simulink model "Vehicle_Dynamics_Testrig"  (R2025a)
settings: Solver=ode23t  StartTime=0.0  StopTime=400  RelTol=1e-3  AbsTol=1e-4  EnableMultiTasking=on
PostLoadFcn:
  | warning off Simulink:Engine:SaveWithDisabledLinks_Warning
  | warning off Simulink:Engine:UsingDefaultMaxStepSize
undefined symbols (not defined in the file): DCT_Param, sigbuilder_block
libraries: fl_lib x22, nesl_utility x6, DCT_Vehicle_Dynamics_Lib x1, sdl_lib x1
Description:
  | Copyright 2014-2025 The MathWorks, Inc.
settings Model: Creator=smiller  LastModifiedBy=smiller
settings SolverCC: AutoScaleAbsTol=off  AlgebraicLoopSolver=TrustRegion
settings DataIOCC: LimitDataPoints=on  SaveFormat=Array  SignalLoggingSaveFormat=ModelDataLogs  ReturnWorkspaceOutputs=off
settings OptimizationCC: ReuseModelBlockBuffer=off  ExpressionDepthLimit=2147483647.0  LifeSpan=inf
settings DebuggingCC: UnderspecifiedInitializationDetection=Classic  MergeDetectMultiDrivingBlocksExec=none  SolverPrmCheckMsg=warning  FcnCallInpInsideContextMsg=warning  UnconnectedInputMsg=warning  UnconnectedOutputMsg=warning  UnconnectedLineMsg=warning  AllowSymbolicDim=off  StateNameClashWarn=warning  PregeneratedLibrarySubsystemCodeDiagnostic=none  SFUnexpectedBacktrackingDiag=warning  SFNoUnconditionalDefaultTransitionDiag=warning  SFExecutionAtInitializationDiag=none  ArithmeticOperatorsInVariantConditions=warning
settings HardwareCC: ProdBitPerPointer=32.0  ProdBitPerSizeT=32.0  ProdBitPerPtrDiffT=32.0  ProdLargestAtomicFloat=None  ProdIntDivRoundTo=Undefined  ProdEndianess=Unspecified  ProdWordSize=32.0  ProdHWDeviceType=32-bit Generic
settings ModelReferenceCC: EnableRefExpFcnMdlSchedulingChecks=on  PropagateSignalLabelsOutOfModel=off
settings SFSimCC: SimUseLocalCustomCode=off  CustomCodeUndefinedFunction=UseInterfaceOnly
settings RTWCC: RTWUseLocalCustomCode=off  GPUComputeCapability=3.5  DLArmComputeVersion=19.05
settings CodeAppCC: StateflowObjectComments=on
settings GRTTargetCC: TargetLangStandard=C89/C90 (ANSI)  CombineOutputUpdateFcns=off  GRTInterface=on
settings ConfigComp: CovMetricSettings=dw  CovSaveCumulativeToWorkspaceVar=on  CovSaveSingleToWorkspaceVar=on  CovExternalEMLEnable=off  CovSFcnEnable=off
settings SimscapeCC: SimscapeNormalizeSystem=off  SimscapeNominalValues="[{\"value\":\"10\",\"unit\":\"V\"},{\"value\":\"1\",\"unit\":\"A\"},{\"value\":\"10\",\"unit\":\"N*m\"},{\"value\":\"10\",\"unit\":\"bar\"},{\"value\":\"100\",\"unit\":\"kJ/kg\"},{\"value\":\"1\",\"unit\":\"kW\"},{\"value\":\"300\",\"unit\":\"K\"},{\"value\":\"100\",\"unit\":\"cm^3/s\"},{\"value\":\"1\",\"unit\":\"kN\"},{\"value\":\"1\",\"unit\":\"g/cm^3\"},{\"value\":\"1\",\"unit\":\"l\"},{\"value\":\"1\",\"unit\":\"cm^2\"},{\"value\":\"60\",\"unit\":\"Hz\"}]"

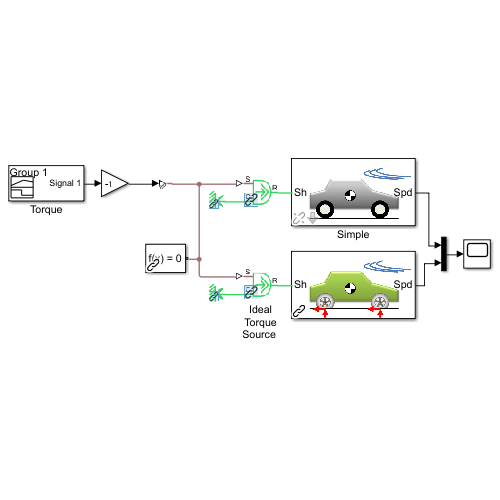
[thumbnail: Simulink's stored preview of the top-level diagram]
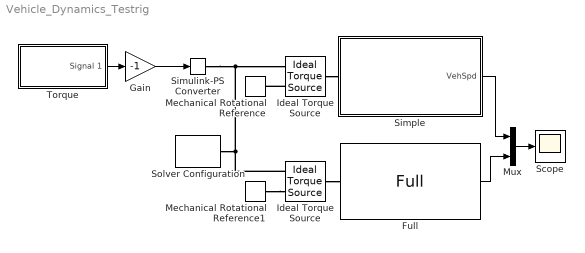
== system Vehicle_Dynamics_Testrig ==
  Full : DCT_Vehicle_Dynamics_Lib/Full  SystemSampleTime=-1  VariantActivationTime=update diagram  EmptyChoice=off  PassThrough=off  PassThroughVariantControl=(default)  EmptyChoiceVariantControl=(default)  AllowFlexibleInterface=on  Latency=0  AutoFrameSizeCalculation=off
  Gain : Gain  Gain=-1
  Ideal Torque Source : fl_lib/Mechanical/Mechanical Sources/Ideal Torque Source
  "Ideal Torque Source " : fl_lib/Mechanical/Mechanical Sources/Ideal Torque Source
  Mechanical Rotational Reference : fl_lib/Mechanical/Rotational Elements/Mechanical Rotational Reference
  Mechanical Rotational Reference1 : fl_lib/Mechanical/Rotational Elements/Mechanical Rotational Reference
  Mux : Mux  Inputs=2
  Scope : Scope
      settings: TimeSpan=400  ActiveDisplayYMinimum=-12.14127  ActiveDisplayYMaximum=109.27138
  Simple : Subsystem  AncestorBlock=DCT_Vehicle_Dynamics_Lib/Simple  mask(Rigid vehicle model){mass=DCT_Param.Vehicle.Mass, area=DCT_Param.Vehicle.Frontal_Area, Cd=DCT_Param.Vehicle.Aero_Drag_Coeff, radius=DCT_Param.Vehicle.Tire.Radius, wheel_inertia=DCT_Param.Vehicle.Tire.Inertia, gear_ratio=DCT_Param.Vehicle.Final_Drive_Ratio}
      mask prompts: mass "Vehicle mass (Kg)"; area "Vehicle Area (m^2)"; Cd "Aerodynamic drag coefficient (unitless)"; radius "Tire radius (m)"; wheel_inertia "Total wheel inertia (kg*m^2)"; gear_ratio "Engine to vehicle gear ratio"
      mask help: Model vehicle effective inertia and drag force as seen by the engine. It is assumed that the vehicle is moving on flat terrain. No bearing friction or gear losses are included.
      mask init:
      | gravity = 9.81;
      settings: LibrarySourceBlock=DCT_Vehicle_Dynamics_Lib/Simple
      mask Display:
      | image(imread('DCT_Vehicle_Dynamics_Simple_IMAGE.jpg'));
      | port_label('LConn',1,'Sh');
      | port_label('output',1,'Spd');
  Simulink-PS Converter : nesl_utility/Simulink-PS Converter  PhysicalDomain=network_engine_domain  SubClassName=ps_input  LeftPortType=input  RightPortType=output  PseudoPeriodic=off  Frequencies=[]  NoiseDistribution=none  NoiseParameters=[]  Unit=1  AffineConversion=off  FilteringAndDerivatives=zero  SimscapeFilterOrder=1  InputFilterTimeConstant=0.005  UdotUserProvided=0
  Solver Configuration : nesl_utility/Solver Configuration  PhysicalDomain=network_engine_domain  SubClassName=solver  LeftPortType=input  RightPortType=generic  Tones=[]  Harmonics=[]  SimulateNoise=off  Profile=off  UseLocalSampling=off  EnableSwitchedLinearOptims=on  FrequencyDomain=off  UseCCode=off  RelTol=0.001  AbsTol=1e-06  MinStep=1e-09  ToWorkspace=off  RevertToSquareIcSolve=off  NumHomotopyIterations=100  PhasorMode=off  PhasorModeNumHarmonics=1  ConsistencySolver=NEWTON_FTOL  IndexReductionMethod=DerivativeReplacement  DoDC=off  ResidualTolerance=1e-9  ConsistencyTolSource=GLOBAL  ConsistencyAbsTol=0.001  ConsistencyRelTol=0.001  ConsistencyTolFactor=0.001  UseLocalSolver=off  LocalSolverChoice=NE_BACKWARD_EULER_ADVANCER  ResolveIndetEquations=on  FunctionEvalNumThread=1  LocalSolverSampleTime=.001  DoFixedCost=off  MaxNonlinIter=3  MaxModeIter=2  ComputeImpulses=off  ImpulseIterations=2  LinearAlgebra=Sparse  LinearAlgebraNumThread=0  EquationFormulation=NE_TIME_EF  DelaysMemoryBudget=1024  AutomaticFiltering=on  FilteringTimeConstant=0.001  PartitionStorageMethod=AS_NEEDED  PartitionMemoryBudget=1024  PartitionMethod=FAST  MultibodyUseLocalSolver=off  MultibodyLocalSolverChoice=ODE1  MultibodyLocalSolverSampleTime=0.001
  Torque : Subsystem  Tag=STV Subsys  LoadFcn=sigbuilder_block('load');  StartFcn=sigbuilder_block('start');  StopFcn=sigbuilder_block('stop');  ClipboardFcn=sigbuilder_block('clipboard');  mask(Sigbuilder block){tuvar=[0:10]}
      mask help: Create and generate interchangeable groups of signals whose waveforms are piecewise linear.
      mask init:
      | if ~strcmp(get_param(bdroot(gcbh),'SimulationStatus'),'stopped') tuvar = sigbuilder_block('maskInit'); end
      settings: CopyFcn=sigbuilder_block('copy');  DeleteFcn=sigbuilder_block('delete');  ModelCloseFcn=sigbuilder_block('modelClose');  PreSaveFcn=sigbuilder_block('preSave');  PauseFcn=sigbuilder_block('pause')  ContinueFcn=sigbuilder_block('continue')  NameChangeFcn=sigbuilder_block('namechange');  OpenFcn=sigbuilder_block('open',[437.25 199.5 550.5 399.75 ]);  CloseFcn=sigbuilder_block('close');
      mask Display: plot(0, 0, 100, 100,[2, 2, 32, 32, 2], [68, 8, 8, 68, 68],[32, 2], [38, 38], [32, 19, 2],[53, 60, 44], [32, 17, 17, 2],[16, 16, 31, 31]);txt = getActiveGroup(gcbh);text(2, 100, txt,'verticalAlignment', 'top');
  wires:
  Simple/1(VehSpd) -> Mux/1
  Mux/1 -> Scope/1
  Full/1 -> Mux/2
  Torque/1(Signal 1) -> Gain/1
  Gain/1 -> Simulink-PS Converter/1
  connections:
  Ideal Torque Source/LConn1 -- Simple/LConn1
  Ideal Torque Source/RConn2 -- Mechanical Rotational Reference/LConn1
  "Ideal Torque Source "/RConn1 -- Ideal Torque Source/RConn1 -- Simulink-PS Converter/RConn1 -- Solver Configuration/RConn1
  Mechanical Rotational Reference1/LConn1 -- "Ideal Torque Source "/RConn2
  "Ideal Torque Source "/LConn1 -- Full/LConn1

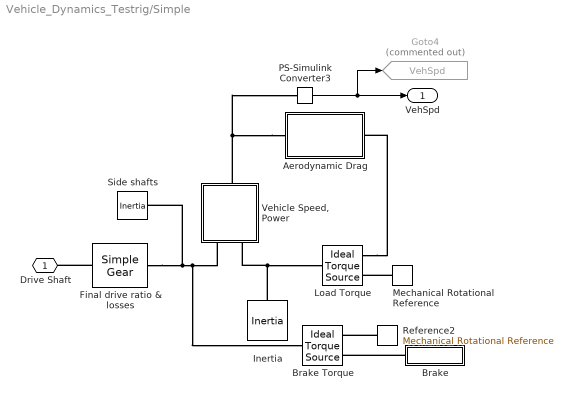
== system Vehicle_Dynamics_Testrig/Simple ==
  Aerodynamic Drag : Subsystem
  Brake : Subsystem
  Brake Torque : fl_lib/Mechanical/Mechanical Sources/Ideal Torque Source
  Final drive ratio & losses : sdl_lib/Gears/Simple Gear  ratio=gear_ratio  rotation_direction=3-2*(2)  friction_model=1  T_noload=0.1 N*m  T_nom=5 N*m  efficiency_nom=0.8  efficiency=DCT_Param.Vehicle.Final_Drive_Efficiency  temperature_TLU=[ 280 300 320 ] K  load_TLU=[ 1 5 10 ] N*m  efficiency_TLU=[ 0.95 0.9 0.85 ]  efficiency_TLU2=[ 0.85 0.8 0.75; 0.95 0.9 0.85; 0.85 0.8 0.7 ]  w_thr=DCT_Param.Vehicle.Final_Drive_Vel_Thresh rad/s  pwr_thr=0.001 W  enable_backlash=false  hardstop_model=simscape.enum.hardstop.smooth  backlash_distance=1e-3 mm  r_base=0.1 m  transition=1e-4 mm  backlash_stiffness=1e7 N/m  backlash_damping=1e6 N*s/m  coeff_rest=0  v_tol=0.001 m/s  f_tol=0 N  mu_visc=[0 0] N*m/(rad/s)  thermal_mass=50 J/K  temperature_specify=off  temperature_priority=High  temperature=300 K  temperature_nominal_specify=off  temperature_nominal_value=1  temperature_nominal_unit=K  x_backlash_specify=off  x_backlash_priority=None  x_backlash=0 mm  x_backlash_nominal_specify=off  x_backlash_nominal_value=1  x_backlash_nominal_unit=mm  f_hardstop_specify=off  f_hardstop_priority=None  f_hardstop=0 N  f_hardstop_nominal_specify=off  f_hardstop_nominal_value=1  f_hardstop_nominal_unit=N  v_backlash_specify=off  v_backlash_priority=None  v_backlash=0 m/s  v_backlash_nominal_specify=off  v_backlash_nominal_value=1  v_backlash_nominal_unit=m/s
  Goto4 : Goto  Commented=on  GotoTag=VehSpd  TagVisibility=global
  Inertia : fl_lib/Mechanical/Rotational Elements/Inertia  inertia=mass*radius*radius kg*m^2  num_ports=foundation.enum.numPorts2.one  w_specify=on  w_priority=High  w=0 rad/s  w_nominal_specify=off  w_nominal_value=1  w_nominal_unit=rad/s  t_specify=off  t_priority=High  t=0 N*m  t_nominal_specify=off  t_nominal_value=1  t_nominal_unit=N*m
  Load Torque : fl_lib/Mechanical/Mechanical Sources/Ideal Torque Source
  Mechanical Rotational Reference : fl_lib/Mechanical/Rotational Elements/Mechanical Rotational Reference
  PS-Simulink Converter3 : nesl_utility/PS-Simulink Converter  PhysicalDomain=network_engine_domain  SubClassName=ps_output  LeftPortType=input  RightPortType=output  PseudoPeriodic=off  Frequencies=[]  VectorFormat=1-D array  Unit=km/hr  AffineConversion=off
  Reference2 : fl_lib/Mechanical/Rotational Elements/Mechanical Rotational Reference
  Side shafts : fl_lib/Mechanical/Rotational Elements/Inertia  inertia=DCT_Param.Vehicle.Side_Shaft_Inertia+2*wheel_inertia kg*m^2  num_ports=foundation.enum.numPorts2.one  w_specify=on  w_priority=High  w=DCT_Param.Vehicle.Side_Shaft_Initial_Velocity rad/s  w_nominal_specify=off  w_nominal_value=1  w_nominal_unit=rad/s  t_specify=off  t_priority=High  t=0 N*m  t_nominal_specify=off  t_nominal_value=1  t_nominal_unit=N*m
  "Vehicle Speed, Power" : Subsystem
  Drive Shaft : PMIOPort  Side=Left
  VehSpd : Outport  VectorParamsAs1DForOutWhenUnconnected=off
  wires:
  PS-Simulink Converter3/1 -> Goto4/1, VehSpd/1
  connections:
  Reference2/LConn1 -- Brake Torque/RConn2
  Brake/RConn1 -- Brake Torque/RConn1
  Side shafts/LConn1 -- Brake Torque/LConn1 -- "Vehicle Speed, Power"/LConn1 -- Final drive ratio & losses/RConn1
  "Vehicle Speed, Power"/LConn2 -- Inertia/LConn1 -- Load Torque/LConn1
  Mechanical Rotational Reference/LConn1 -- Load Torque/RConn2
  Load Torque/RConn1 -- Aerodynamic Drag/RConn1
  Aerodynamic Drag/LConn1 -- "Vehicle Speed, Power"/RConn1 -- PS-Simulink Converter3/LConn1
  Final drive ratio & losses/LConn1 -- Drive Shaft/RConn1

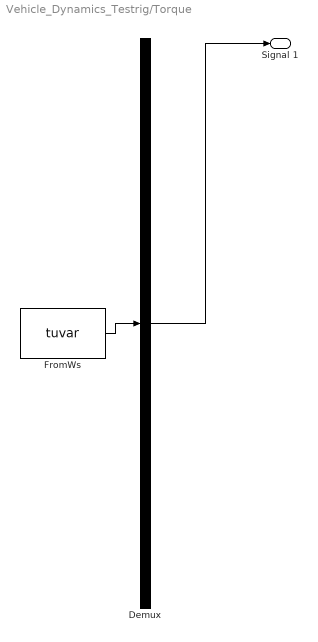
== system Vehicle_Dynamics_Testrig/Torque ==
  Demux : Demux  Tag=STV Demux  Outputs=1
      settings: DisplayOption=none
  FromWs : FromWorkspace  Tag=STV FromWs  VariableName=tuvar
      SigBuilderData=|
      | common.afterFinalStr = 'Extrapolate'
      | common.sampleTime = 0
      | dataSet.timeRange = [0 400]
      | dataSet.name = 'Group 1'
      | sbobj.Groups.Name = 'Group 1'
      | sbobj.Groups.Signals.Name = 'Signal 1'
      | sbobj.Groups.Signals.XData = [0 6 6 50 50 150 150 170 170 400]
      | sbobj.Groups.Signals.YData = [0 0 100 100 0 0 100 100 0 0]
      | sbobj.Groups.TimeRange = [0 400]
  Signal 1 : Outport  Tag=STV Outport  VectorParamsAs1DForOutWhenUnconnected=off
  wires:
  Demux/1 -> Signal 1/1
  FromWs/1 -> Demux/1

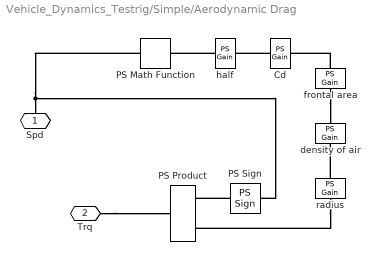
== system Vehicle_Dynamics_Testrig/Simple/Aerodynamic Drag ==
  Cd : fl_lib/Physical Signals/Functions/PS Gain  gain=Cd
  PS Math Function : fl_lib/Physical Signals/Functions/PS Math Function  fcn_choice=7  v=1
  PS Product : fl_lib/Physical Signals/Functions/PS Product
  PS Sign : fl_lib/Physical Signals/Nonlinear Operators/PS Sign
      settings: InternalSimscapePortConfiguration="{\"Bottom\":[],\"Left\":[{\"id\":\"I\",\"label\":\"\",\"type\":\"input\"}],\"Right\":[{\"id\":\"O\",\"label\":\"\",\"type\":\"output\"}],\"Top\":[]}"
  density of air : fl_lib/Physical Signals/Functions/PS Gain  gain=1.2 kg/m^3
  frontal area : fl_lib/Physical Signals/Functions/PS Gain  gain=area m^2
  half : fl_lib/Physical Signals/Functions/PS Gain  gain=1/2
  radius : fl_lib/Physical Signals/Functions/PS Gain  gain=-radius m
  Spd : PMIOPort  Side=Left
  Trq : PMIOPort  Port=2  Side=Right
  connections:
  Trq/RConn1 -- PS Product/RConn1
  Spd/RConn1 -- PS Sign/LConn1 -- PS Math Function/LConn1
  half/LConn1 -- PS Math Function/RConn1
  Cd/LConn1 -- half/RConn1
  radius/RConn1 -- PS Product/LConn1
  PS Sign/RConn1 -- PS Product/LConn2
  radius/LConn1 -- density of air/RConn1
  frontal area/LConn1 -- Cd/RConn1
  frontal area/RConn1 -- density of air/LConn1

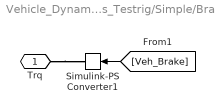
== system Vehicle_Dynamics_Testrig/Simple/Brake ==
  Simulink-PS Converter1 : nesl_utility/Simulink-PS Converter  PhysicalDomain=network_engine_domain  SubClassName=ps_input  LeftPortType=input  RightPortType=output  PseudoPeriodic=off  Frequencies=[]  NoiseDistribution=none  NoiseParameters=[]  Unit=1  AffineConversion=off  FilteringAndDerivatives=zero  SimscapeFilterOrder=1  InputFilterTimeConstant=0.005  UdotUserProvided=0
  Trq : PMIOPort  Side=Right
  wires:
  [Veh_Brake] -> Simulink-PS Converter1/1
  connections:
  Trq/RConn1 -- Simulink-PS Converter1/RConn1

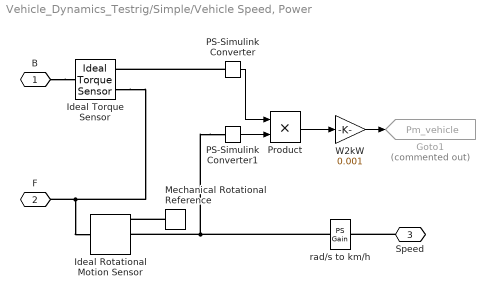
== system Vehicle_Dynamics_Testrig/Simple/Vehicle Speed, Power ==
  Goto1 : Goto  Commented=on  GotoTag=Pm_vehicle  TagVisibility=global
  Ideal Rotational Motion Sensor : fl_lib/Mechanical/Mechanical Sensors/Ideal Rotational Motion Sensor  reference=foundation.enum.MeasurementReference.difference  acceleration_port=false  velocity_port=true  position_port=true  wrap_angle=simscape.enum.onoff.off  offset=0 rad
  Ideal Torque Sensor : fl_lib/Mechanical/Mechanical Sensors/Ideal Torque Sensor
  Mechanical Rotational Reference : fl_lib/Mechanical/Rotational Elements/Mechanical Rotational Reference
  PS-Simulink Converter : nesl_utility/PS-Simulink Converter  PhysicalDomain=network_engine_domain  SubClassName=ps_output  LeftPortType=input  RightPortType=output  PseudoPeriodic=off  Frequencies=[]  VectorFormat=1-D array  Unit=N*m  AffineConversion=off
  PS-Simulink Converter1 : nesl_utility/PS-Simulink Converter  PhysicalDomain=network_engine_domain  SubClassName=ps_output  LeftPortType=input  RightPortType=output  PseudoPeriodic=off  Frequencies=[]  VectorFormat=1-D array  Unit=rad/s  AffineConversion=off
  Product : Product  RndMeth=Zero
  W2kW : Gain  Gain=0.001
  rad/s to km/h : fl_lib/Physical Signals/Functions/PS Gain  gain=radius*3.6 (km/hr)/(rad/s)
  B : PMIOPort  Side=Left
  F : PMIOPort  Port=2  Side=Left
  Speed : PMIOPort  Port=3  Side=Right
  wires:
  PS-Simulink Converter1/1 -> Product/2
  PS-Simulink Converter/1 -> Product/1
  Product/1 -> W2kW/1
  W2kW/1 -> Goto1/1
  connections:
  Speed/RConn1 -- rad/s to km/h/RConn1
  PS-Simulink Converter1/LConn1 -- Ideal Rotational Motion Sensor/RConn2 -- rad/s to km/h/LConn1
  PS-Simulink Converter/LConn1 -- Ideal Torque Sensor/RConn2
  B/RConn1 -- Ideal Torque Sensor/LConn1
  Ideal Torque Sensor/RConn1 -- F/RConn1 -- Ideal Rotational Motion Sensor/LConn1
  Mechanical Rotational Reference/LConn1 -- Ideal Rotational Motion Sensor/RConn1
